simulink model "single_phase_full_controlled_rectifier_circuit"  (R2024a)
settings: Solver=VariableStepAuto  StartTime=0.0  StopTime=10.0  RelTol=1e-3
libraries: spsThyristorLib x4, spsACVoltageSourceLib x1, spsMeanPhasorLib x1, spsVoltageMeasurementLib x1, spspowerguiLib x1
settings Model: Creator=haris  LastModifiedBy=haris
settings RTWCC: GPUComputeCapability=3.5

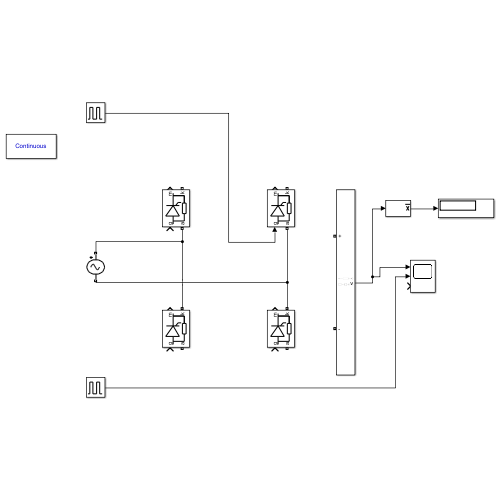
[thumbnail: Simulink's stored preview of the top-level diagram]
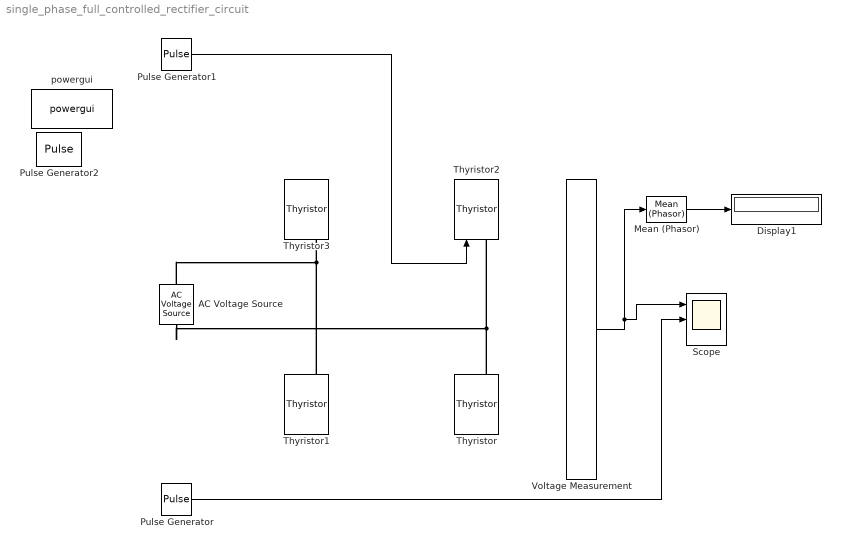
== system single_phase_full_controlled_rectifier_circuit ==
  AC Voltage Source : spsACVoltageSourceLib/AC Voltage Source  Amplitude=100  Phase=0  Frequency=60  SampleTime=0  Measurements=None  BusType=swing  Pref=10e3  Qref=0  Qmin=-inf  Qmax=+inf
  Display1 : Display
  Mean (Phasor) : spsMeanPhasorLib/Mean (Phasor)  Freq=60  Vinit=0  Ts=0
      settings: LibrarySourceBlock=|
      | sps_lib/Sensors and Measurements/Mean
      | (Phasor)
  Pulse Generator : DiscretePulseGenerator  PulseType=Time based  Period=10  PulseWidth=5
  Pulse Generator1 : DiscretePulseGenerator  PulseType=Time based  Period=10  PulseWidth=5
  Scope : Scope  NumInputPorts=3
  Thyristor{,1..3} (4 alike) : spsThyristorLib/Thyristor  Ron=0.001  Lon=0  Vf=0.8  IC=0  Rs=500  Cs=250e-9  Measurements=on
  Voltage Measurement : spsVoltageMeasurementLib/Voltage Measurement  PhasorSimulation=off  OutputType=Complex  PSBequivalent=0
  powergui : spspowerguiLib/powergui  Priority=1  SimulationMode=Continuous  SampleTime=50e-6  frequency=60  Iterations=50  frequencyindice=60  Pbase=100e6  ErrMax=1e-4  UnitsV=kV  UnitsW=MW  buscounter=0  FunctionMessages=off  echomessages=off  EnableUseOfTLC=off  CurrentSourceSwitches=off  DisableSnubberDevices=off  DisableRonSwitches=off  DisableVfSwitches=off  DisplayEquations=off  AutomaticDiscreteSolvers=off  SolverType=Tustin/Backward Euler (TBE)  Interpol=off  ExternalGateDelay=off  methode=off  Ts=100  x0status=blocks  SPID=on  SwTol=0  HookPort=off  NonlinearTolerance=1e-4  nMaxIteration=100  ContinueOnMaxIteration=off  RestoreLinks=warning  ResistiveCurrentMeasurement=off  Frange=[0:2:500]  Ylog=off  Xlog=on  ShowGrid=off  save=off  variable=ZData  structure=0  ZoomFFT=off  StartTime=0.0  cycles=1  DisplayStyle=1  fundamental=60  FreqAxis=off  MaxFrequency=1000  frequencyindicesteady=1  RmsSteady=1  display=off
  Pulse Generator2 : DiscretePulseGenerator  IOType=siggen  PulseType=Time based  PulseWidth=50
  wires:
  Mean (Phasor)/1 -> Display1/1
  Voltage Measurement/1 -> Mean (Phasor)/1, Scope/1
  Pulse Generator1/1 -> Thyristor2/1
  Pulse Generator/1 -> Scope/2
  connections:
  Thyristor1/RConn1 -- AC Voltage Source/RConn1 -- Thyristor3/LConn1
  Thyristor/RConn1 -- AC Voltage Source/LConn1 -- Thyristor2/LConn1
